simulink model "Shaddad_Plant"  (R2026b)
undefined symbols (not defined in the file): P, Ts
libraries: nesl_utility x1
settings Model: Creator=aomar  LastModifiedBy=aomar

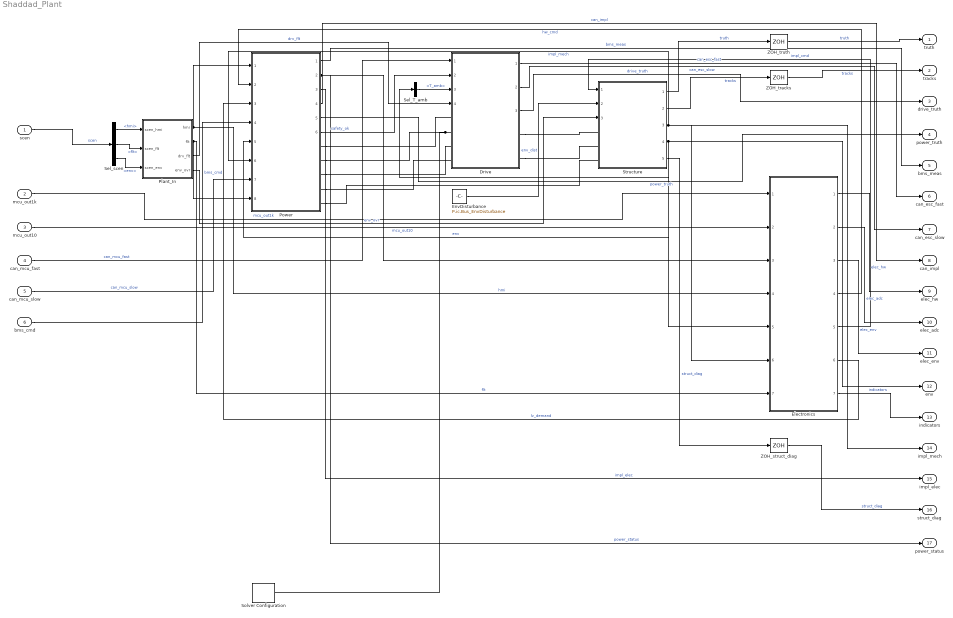
== system Shaddad_Plant ==
  scen : Inport  OutDataTypeStr=Bus: Bus_ScenarioIn  SampleTime=Ts.ctrl  BusOutputAsStruct=on
  mcu_out1k : Inport  Port=2  OutDataTypeStr=Bus: Bus_McuOut1k  SampleTime=Ts.base  BusOutputAsStruct=on
  mcu_out10 : Inport  Port=3  OutDataTypeStr=Bus: Bus_McuOut10  SampleTime=Ts.ctrl  BusOutputAsStruct=on
  can_mcu_fast : Inport  Port=4  OutDataTypeStr=Bus: Bus_Can1_McuFast  SampleTime=Ts.ctrl  BusOutputAsStruct=on
  can_mcu_slow : Inport  Port=5  OutDataTypeStr=Bus: Bus_Can1_McuSlow  SampleTime=Ts.comm  BusOutputAsStruct=on
  bms_cmd : Inport  Port=6  OutDataTypeStr=Bus: Bus_BMS_Cmd  SampleTime=Ts.ctrl  BusOutputAsStruct=on
  Drive : Subsystem  ReferencedSubsystem=drive_system
  Electronics : Subsystem  ReferencedSubsystem=Electronics_Plant
  EnvDisturbance : Constant  Value=P.ic.Bus_EnvDisturbance  OutDataTypeStr=Bus: Bus_EnvDisturbance  SampleTime=Ts.base
  Plant_In : Subsystem
  Power : Subsystem  ReferencedSubsystem=Power_Plant
  Sel_T_amb : BusSelector  OutputSignals=T_amb
  Sel_scen : BusSelector  OutputSignals=hmi,flt,env
  Solver Configuration : nesl_utility/Solver Configuration  PhysicalDomain=network_engine_domain  SubClassName=solver  LeftPortType=input  RightPortType=generic  Tones=[]  Harmonics=[]  SimulateNoise=off  Profile=off  UseLocalSampling=off  EnableSwitchedLinearOptims=on  FrequencyDomain=off  UseCCode=off  RelTol=0.001  AbsTol=0.001  MinStep=1e-09  ToWorkspace=off  RevertToSquareIcSolve=off  NumHomotopyIterations=100  PhasorMode=off  PhasorModeNumHarmonics=1  ConsistencySolver=NEWTON_XTOL_AFTER_FTOL  CanonicalOrdering=CANONICAL  OptimizeIntermediates=OPTIMIZED  MulticoreSolverChoice=BACKWARD_EULER  IndexReductionMethod=DerivativeReplacement  DoDC=off  ResidualTolerance=1e-09  ConsistencyTolSource=GLOBAL  ConsistencyAbsTol=0.001  ConsistencyRelTol=0.001  ConsistencyTolFactor=0.001  UseLocalSolver=on  LocalSolverChoice=NE_BACKWARD_EULER_ADVANCER  ResolveIndetEquations=on  FunctionEvalNumThread=1  LocalSolverSampleTime=P.sim.ssc.Ts  DoFixedCost=on  MaxNonlinIter=P.sim.ssc.MaxNonlinIter  MaxModeIter=P.sim.ssc.MaxModeIter  ComputeImpulses=off  ImpulseIterations=2  LinearAlgebra=auto  LinearAlgebraNumThread=0  EquationFormulation=NE_TIME_EF  DelaysMemoryBudget=1024  AutomaticFiltering=on  FilteringTimeConstant=0.001  PartitionStorageMethod=AS_NEEDED  PartitionMemoryBudget=1024  PartitionMethod=BALANCED  MultibodyUseLocalSolver=off  MultibodyLocalSolverChoice=ODE1  MultibodyLocalSolverSampleTime=0.001
  Structure : Subsystem  ReferencedSubsystem=structure_plant
  ZOH_struct_diag : ZeroOrderHold  SampleTime=Ts.ctrl
  ZOH_tracks : ZeroOrderHold  SampleTime=Ts.base
  ZOH_truth : ZeroOrderHold  SampleTime=Ts.base
  truth : Outport  OutDataTypeStr=Bus: Bus_TruthState  SampleTime=Ts.base  BusOutputAsStruct=on
  tracks : Outport  Port=2  OutDataTypeStr=Bus: Bus_TrackState  SampleTime=Ts.base  BusOutputAsStruct=on
  drive_truth : Outport  Port=3  OutDataTypeStr=Bus: Bus_DriveTruth  SampleTime=Ts.base  BusOutputAsStruct=on
  power_truth : Outport  Port=4  OutDataTypeStr=Bus: Bus_PowerTruth  SampleTime=Ts.hk  BusOutputAsStruct=on
  bms_meas : Outport  Port=5  OutDataTypeStr=Bus: Bus_BMS_Meas  SampleTime=Ts.ctrl  BusOutputAsStruct=on
  can_esc_fast : Outport  Port=6  OutDataTypeStr=Bus: Bus_Can1_EscFast  SampleTime=Ts.ctrl  BusOutputAsStruct=on
  can_esc_slow : Outport  Port=7  OutDataTypeStr=Bus: Bus_Can1_EscSlow  SampleTime=Ts.comm  BusOutputAsStruct=on
  can_impl : Outport  Port=8  OutDataTypeStr=Bus: Bus_Can1_Impl  SampleTime=Ts.comm  BusOutputAsStruct=on
  elec_hw : Outport  Port=9  OutDataTypeStr=Bus: Bus_ElecHwIn  SampleTime=Ts.base  BusOutputAsStruct=on
  elec_adc : Outport  Port=10  OutDataTypeStr=Bus: Bus_ElecAdc  SampleTime=Ts.comm  BusOutputAsStruct=on
  elec_env : Outport  Port=11  OutDataTypeStr=Bus: Bus_ElecEnv  SampleTime=Ts.hk  BusOutputAsStruct=on
  env : Outport  Port=12  OutDataTypeStr=Bus: Bus_EnvState  SampleTime=Ts.hk  BusOutputAsStruct=on
  indicators : Outport  Port=13  OutDataTypeStr=Bus: Bus_IndicatorOut  SampleTime=Ts.hk  BusOutputAsStruct=on
  impl_mech : Outport  Port=14  OutDataTypeStr=Bus: Bus_ImplMechState  SampleTime=Ts.ctrl  BusOutputAsStruct=on
  impl_elec : Outport  Port=15  OutDataTypeStr=Bus: Bus_ImplElecState  SampleTime=Ts.ctrl  BusOutputAsStruct=on
  struct_diag : Outport  Port=16  OutDataTypeStr=Bus: Bus_StructureDiag  SampleTime=Ts.ctrl  BusOutputAsStruct=on
  power_status : Outport  Port=17  OutDataTypeStr=Bus: Bus_PowerStatus  SampleTime=Ts.base  BusOutputAsStruct=on
  wires:
  scen/1 -> Sel_scen/1  "scen"
  mcu_out1k/1 -> Electronics/1  "mcu_out1k"
  mcu_out10/1 -> Electronics/2  "mcu_out10"
  can_mcu_fast/1 -> Drive/1  "can_mcu_fast"
  can_mcu_slow/1 -> Power/7  "can_mcu_slow"
  bms_cmd/1 -> Power/4  "bms_cmd"
  Sel_scen/1 -> Plant_In/1(scen_hmi)  "<hmi>"
  Sel_scen/2 -> Plant_In/2(scen_flt)  "<flt>"
  Sel_scen/3 -> Plant_In/3(scen_env)  "<env>"
  Plant_In/1(hmi) -> Electronics/4, Power/1  "hmi"
  Plant_In/2(flt) -> Electronics/7, Power/8  "flt"
  Plant_In/3(drv_flt) -> Drive/4  "drv_flt"
  Plant_In/4(env_ovr) -> Structure/3  "env_ovr"
  Power/1 -> bms_meas/1  "bms_meas"
  Power/2 -> power_status/1, Electronics/3  "power_status"
  Power/3 -> impl_elec/1  "impl_elec"
  Power/4 -> can_impl/1  "can_impl"
  Power/5 -> power_truth/1  "power_truth"
  Power/6 -> Drive/2  "safety_ok"
  Sel_T_amb/1 -> Drive/3  "<T_amb>"
  EnvDisturbance/1 -> Structure/2  "env_dist"
  Drive/1 -> can_esc_fast/1  "can_esc_fast"
  Drive/2 -> can_esc_slow/1  "can_esc_slow"
  Drive/3 -> drive_truth/1  "drive_truth"
  Structure/1 -> ZOH_truth/1  "truth"
  Structure/2 -> ZOH_tracks/1  "tracks"
  Structure/5 -> ZOH_struct_diag/1  "struct_diag"
  ZOH_truth/1 -> truth/1  "truth"
  ZOH_tracks/1 -> tracks/1  "tracks"
  ZOH_struct_diag/1 -> struct_diag/1  "struct_diag"
  Electronics/1 -> elec_hw/1  "elec_hw"
  Electronics/2 -> elec_adc/1  "elec_adc"
  Electronics/3 -> elec_env/1  "elec_env"
  Electronics/4 -> Power/2  "hw_cmd"
  Electronics/5 -> Structure/1  "impl_cmd"
  Electronics/6 -> Power/3  "lv_demand"
  Electronics/7 -> indicators/1  "indicators"
  Structure/3 -> impl_mech/1, Electronics/6, Power/6  "impl_mech"
  Structure/4 -> env/1, Electronics/5, Sel_T_amb/1, Power/5  "env"
  connections:
  Power/RConn1 -- Drive/LConn1
  Drive/LConn2 -- Power/RConn2 -- Solver Configuration/RConn1
  Power/RConn3 -- Drive/LConn3
  Power/RConn4 -- Drive/LConn4
  Drive/RConn1 -- Structure/LConn1
  Drive/RConn2 -- Structure/LConn2
  Power/RConn5 -- Structure/LConn3

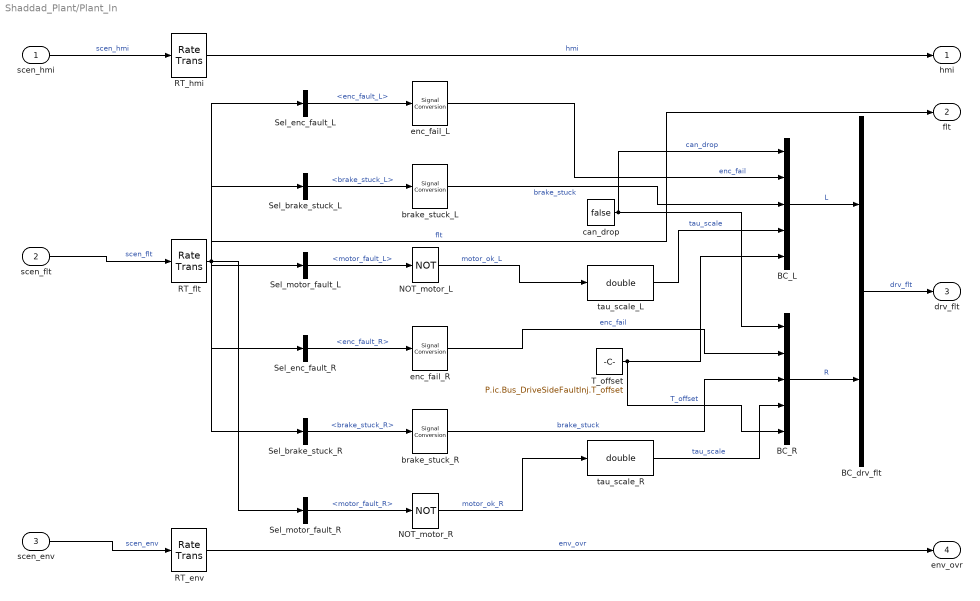
== system Shaddad_Plant/Plant_In ==
  scen_hmi : Inport  OutDataTypeStr=Bus: Bus_HmiInputs  SampleTime=Ts.scen
  scen_flt : Inport  Port=2  OutDataTypeStr=Bus: Bus_FaultInject  SampleTime=Ts.scen
  scen_env : Inport  Port=3  OutDataTypeStr=Bus: Bus_EnvOverride  SampleTime=Ts.scen
  BC_L : BusCreator  Inputs=5  OutDataTypeStr=Bus: Bus_DriveSideFaultInj  NonVirtualBus=on
  BC_R : BusCreator  Inputs=5  OutDataTypeStr=Bus: Bus_DriveSideFaultInj  NonVirtualBus=on
  BC_drv_flt : BusCreator  Inputs=2  OutDataTypeStr=Bus: Bus_DriveFaultInj  NonVirtualBus=on
  NOT_motor_L : Logic  Operator=NOT  AllPortsSameDT=off  OutDataTypeStr=boolean
  NOT_motor_R : Logic  Operator=NOT  AllPortsSameDT=off  OutDataTypeStr=boolean
  RT_env : RateTransition  InitialCondition=P.ic.Bus_EnvOverride  OutPortSampleTime=Ts.env
  RT_flt : RateTransition  InitialCondition=P.ic.Bus_FaultInject  OutPortSampleTime=Ts.base
  RT_hmi : RateTransition  InitialCondition=P.ic.Bus_HmiInputs  OutPortSampleTime=Ts.base
  Sel_brake_stuck_L : BusSelector  OutputSignals=brake_stuck_L
  Sel_brake_stuck_R : BusSelector  OutputSignals=brake_stuck_R
  Sel_enc_fault_L : BusSelector  OutputSignals=enc_fault_L
  Sel_enc_fault_R : BusSelector  OutputSignals=enc_fault_R
  Sel_motor_fault_L : BusSelector  OutputSignals=motor_fault_L
  Sel_motor_fault_R : BusSelector  OutputSignals=motor_fault_R
  T_offset : Constant  Value=P.ic.Bus_DriveSideFaultInj.T_offset  OutDataTypeStr=double  SampleTime=Ts.base
  brake_stuck_L : SignalConversion  OverrideOpt=off
  brake_stuck_R : SignalConversion  OverrideOpt=off
  can_drop : Constant  Value=false  OutDataTypeStr=boolean  SampleTime=Ts.base
  enc_fail_L : SignalConversion  OverrideOpt=off
  enc_fail_R : SignalConversion  OverrideOpt=off
  tau_scale_L : DataTypeConversion  OutDataTypeStr=double  SaturateOnIntegerOverflow=off  RndMeth=Floor
  tau_scale_R : DataTypeConversion  OutDataTypeStr=double  SaturateOnIntegerOverflow=off  RndMeth=Floor
  hmi : Outport  OutDataTypeStr=Bus: Bus_HmiInputs
  flt : Outport  Port=2  OutDataTypeStr=Bus: Bus_FaultInject
  drv_flt : Outport  Port=3  OutDataTypeStr=Bus: Bus_DriveFaultInj
  env_ovr : Outport  Port=4  OutDataTypeStr=Bus: Bus_EnvOverride
  wires:
  scen_hmi/1 -> RT_hmi/1  "scen_hmi"
  scen_flt/1 -> RT_flt/1  "scen_flt"
  scen_env/1 -> RT_env/1  "scen_env"
  RT_hmi/1 -> hmi/1  "hmi"
  RT_flt/1 -> Sel_motor_fault_R/1, Sel_brake_stuck_R/1, Sel_enc_fault_L/1, flt/1, Sel_enc_fault_R/1, Sel_brake_stuck_L/1, Sel_motor_fault_L/1  "flt"
  RT_env/1 -> env_ovr/1  "env_ovr"
  Sel_enc_fault_L/1 -> enc_fail_L/1  "<enc_fault_L>"
  Sel_brake_stuck_L/1 -> brake_stuck_L/1  "<brake_stuck_L>"
  Sel_motor_fault_L/1 -> NOT_motor_L/1  "<motor_fault_L>"
  Sel_enc_fault_R/1 -> enc_fail_R/1  "<enc_fault_R>"
  Sel_brake_stuck_R/1 -> brake_stuck_R/1  "<brake_stuck_R>"
  Sel_motor_fault_R/1 -> NOT_motor_R/1  "<motor_fault_R>"
  NOT_motor_L/1 -> tau_scale_L/1  "motor_ok_L"
  NOT_motor_R/1 -> tau_scale_R/1  "motor_ok_R"
  enc_fail_L/1 -> BC_L/2  "enc_fail"
  brake_stuck_L/1 -> BC_L/3  "brake_stuck"
  enc_fail_R/1 -> BC_R/2  "enc_fail"
  brake_stuck_R/1 -> BC_R/3  "brake_stuck"
  can_drop/1 -> BC_R/1, BC_L/1  "can_drop"
  T_offset/1 -> BC_L/5, BC_R/5  "T_offset"
  tau_scale_L/1 -> BC_L/4  "tau_scale"
  tau_scale_R/1 -> BC_R/4  "tau_scale"
  BC_L/1 -> BC_drv_flt/1  "L"
  BC_R/1 -> BC_drv_flt/2  "R"
  BC_drv_flt/1 -> drv_flt/1  "drv_flt"
